simulink model "ex1s"  (R2022a)
settings: Solver=VariableStepAuto  StartTime=0.0  StopTime=10.0  RelTol=1e-3
settings Model: Creator=giova  LastModifiedBy=giova

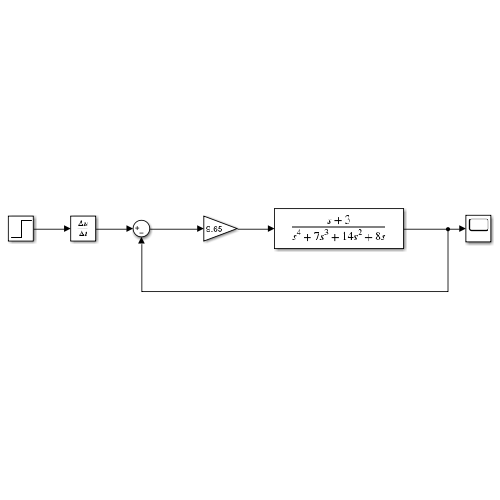
[thumbnail: Simulink's stored preview of the top-level diagram]
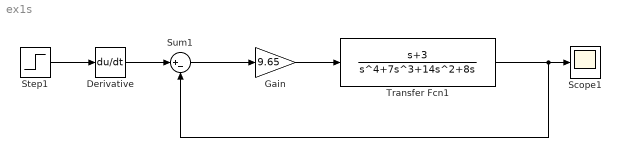
== system ex1s ==
  Derivative : Derivative
  Gain : Gain  Gain=9.65
  Scope1 : Scope
  Step1 : Step  SampleTime=0
  Sum1 : Sum  Inputs=|+-
  Transfer Fcn1 : TransferFcn  Numerator=[1 3]  Denominator=[1 7 14 8 0]
  wires:
  Transfer Fcn1/1 -> Sum1/2, Scope1/1
  Step1/1 -> Derivative/1
  Sum1/1 -> Gain/1
  Gain/1 -> Transfer Fcn1/1
  Derivative/1 -> Sum1/1
